simulink library "Lib_Piccolo"  (R2018b)
settings: Solver=VariableStepAuto  StartTime=0.0  StopTime=10.0  RelTol=1e-3
values from neighbouring files (symbols this model uses):
  AccelErrInt2Brakes = 0.15    [SimulationControlConfig16P.m]    (also in SimulationControlConfig16P_LEGACY.m; SimulationControlConfigTAILLESS.m = 0.2; SimulationControlConfigUTAIL.m = 0.2)
  AileronMax = 25    [SimulationControlConfig16P.m]    (also in SimulationControlConfig16P_LEGACY.m; SimulationControlConfigTAILLESS.m; SimulationControlConfigUTAIL.m)
  AileronPower = 0.00268    [SimulationControlConfig16P.m]    (also in SimulationControlConfig16P_LEGACY.m; SimulationControlConfigTAILLESS.m; SimulationControlConfigUTAIL.m)
  AileronSurfaceMax = 45    [SimulationControlConfig16P.m]    (also in SimulationControlConfig16P_LEGACY.m)
  AileronTrim = 0    [SimulationControlConfig16P.m]    (also in SimulationControlConfig16P_LEGACY.m; SimulationControlConfigTAILLESS.m; SimulationControlConfigUTAIL.m)
  Alt = 1000 + TerrainHeight    [SimulationStateConfig.m]
  AltCruise_m = testPlans(testIndx).terrainElevation * 0.3048 + 200    [SimulationControlConfig16P.m]    (also in SimulationControlConfigTAILLESS.m = 1083; SimulationControlConfigUTAIL.m = testPlans(testIndx).terrainElevation * 0.3048 + 152)
  AltitudeRate2PitchCmdIntegratorInit = 0.1    [SimulationControlPre.m]
  AltMax = 10000    [SimulationControlConfig16P.m]    (also in SimulationControlConfig16P_LEGACY.m; SimulationControlConfigTAILLESS.m; SimulationControlConfigUTAIL.m)
  AltMaxAccel = 1.25    [SimulationControlConfig16P.m]    (also in SimulationControlConfig16P_LEGACY.m = 0.9; SimulationControlConfigTAILLESS.m = 1.7; SimulationControlConfigUTAIL.m = 2)
  AltMin = 0    [SimulationControlConfig16P.m]    (also in SimulationControlConfig16P_LEGACY.m; SimulationControlConfigTAILLESS.m; SimulationControlConfigUTAIL.m)
  AltRateCmd2Pitch = 0.50    (= 0.5)    [SimulationControlConfig16P.m]    (also in SimulationControlConfig16P_LEGACY.m = 0.6; SimulationControlConfigTAILLESS.m = 0.2; SimulationControlConfigUTAIL.m = 0.3)
  AltRateError2Pitch = 0.40    (= 0.4)    [SimulationControlConfig16P.m]    (also in SimulationControlConfig16P_LEGACY.m; SimulationControlConfigTAILLESS.m = 0.55; SimulationControlConfigUTAIL.m = 0.55)
  AltRateErrorInt2Pitch = 0.50    (= 0.5)    [SimulationControlConfig16P.m]    (also in SimulationControlConfig16P_LEGACY.m = 0.45; SimulationControlConfigTAILLESS.m; SimulationControlConfigUTAIL.m = 0.75)
  AltRateLpfCutOff = 3    [SimulationControlConfig16P.m]    (also in SimulationControlConfig16P_LEGACY.m; SimulationControlConfigTAILLESS.m = 2; SimulationControlConfigUTAIL.m = 2)
  AutoNosegear2Rudder = 26    [SimulationControlConfig16P.m]    (also in SimulationControlConfig16P_LEGACY.m; SimulationControlConfigTAILLESS.m = 25.2; SimulationControlConfigUTAIL.m = 14)
  b = 5.54    [SimulationControlConfig16P.m]    (also in SimulationControlConfig16P_LEGACY.m; SimulationControlConfigTAILLESS.m = 2.37; SimulationControlConfigUTAIL.m = 2.37)
  Bank2AileronIntegratorInit = 0    [SimulationControlPre.m]
  BankMax_User = BankMax_User/180*pi    (= 0.523598775598)    [SimulationControlConfig16P.m]    (also in SimulationControlConfig16P_LEGACY.m; SimulationControlConfigTAILLESS.m = 0.610865238198; SimulationControlConfigUTAIL.m = 0.628318530718)
  baseLegFlaps = 20    [SimulationControlConfig16P.m]    (also in SimulationControlConfig16P_LEGACY.m = 0; SimulationControlConfigTAILLESS.m = 15; SimulationControlConfigUTAIL.m = 10)
  C = GeneticOpt.C    [SimulationCostFunction.m]
  c = Sw/b    (= 0.841696750903)    [SimulationControlConfig16P.m]    (also in SimulationControlConfig16P_LEGACY.m; SimulationControlConfigTAILLESS.m = 0.354008438819; SimulationControlConfigUTAIL.m = 0.354008438819)
  cell2WheelFactorMG = 5.98    [SimulationSensorConfig16P_LEGACY.m]
  cell2WheelFactorNG = 1    [SimulationSensorConfig16P_LEGACY.m]
  cellSatMaxMG = 15000    [SimulationSensorConfig16P.m]    (also in SimulationSensorConfig16P_LEGACY.m; SimulationSensorConfigTAILLESS7P.m; SimulationSensorConfigUTAIL7P.m)
  cellSatMaxNG = 1000    [SimulationSensorConfig16P.m]    (also in SimulationSensorConfig16P_LEGACY.m; SimulationSensorConfigTAILLESS7P.m; SimulationSensorConfigUTAIL7P.m)
  cellSatMinMG = -15000    [SimulationSensorConfig16P.m]    (also in SimulationSensorConfig16P_LEGACY.m; SimulationSensorConfigTAILLESS7P.m; SimulationSensorConfigUTAIL7P.m)
  cellSatMinNG = -1000    [SimulationSensorConfig16P.m]    (also in SimulationSensorConfig16P_LEGACY.m; SimulationSensorConfigTAILLESS7P.m; SimulationSensorConfigUTAIL7P.m)
  CL_Limit = CL_Max    (= 0.54)    [SimulationControlConfig16P.m]    (also in SimulationControlConfig16P_LEGACY.m; SimulationControlConfigTAILLESS.m; SimulationControlConfigUTAIL.m = 0.53)
  CL_Max = 0.54    [SimulationControlConfig16P.m]    (also in SimulationControlConfig16P_LEGACY.m; SimulationControlConfigTAILLESS.m; SimulationControlConfigUTAIL.m = 0.53)
  CL_Max_Nom = 0.465    [SimulationControlConfig16P.m]    (also in SimulationControlConfig16P_LEGACY.m; SimulationControlConfigTAILLESS.m = 0.39; SimulationControlConfigUTAIL.m)
  CL_Min = 0    [SimulationControlConfig16P.m]    (also in SimulationControlConfig16P_LEGACY.m; SimulationControlConfigTAILLESS.m; SimulationControlConfigUTAIL.m)
  ClimbMaxFraction = 0.35    [SimulationControlConfig16P.m]    (also in SimulationControlConfig16P_LEGACY.m = 0.24; SimulationControlConfigTAILLESS.m = 0.19; SimulationControlConfigUTAIL.m = 0.21)
  ClimboutMaxBank = 7.0    (= 7)    [SimulationControlConfig16P.m]    (also in SimulationControlConfig16P_LEGACY.m; SimulationControlConfigTAILLESS.m = 5; SimulationControlConfigUTAIL.m)
  ClimboutTimer = 7.0    (= 7)    [SimulationControlConfig16P.m]    (also in SimulationControlConfig16P_LEGACY.m; SimulationControlConfigTAILLESS.m; SimulationControlConfigUTAIL.m)
  dCl_per_dFlap = 0.005581818    [SimulationControlConfig16P.m]    (also in SimulationControlConfig16P_LEGACY.m = 0; SimulationControlConfigTAILLESS.m = 0; SimulationControlConfigUTAIL.m = 0)
  DecelerationCmd = 3.1    [SimulationControlConfig16P.m]    (also in SimulationControlConfig16P_LEGACY.m; SimulationControlConfigTAILLESS.m = 0.1; SimulationControlConfigUTAIL.m = 0.1)
  DeRotateLogicEndTimer = abs((NoseDownLimit_Deg-1)/DeRotateRamp_Dps)    [SimulationControlConfig16P.m]    (also in SimulationControlConfig16P_LEGACY.m; SimulationControlConfigTAILLESS.m; SimulationControlConfigUTAIL.m)
  DeRotateLogicHoldNoseUpTimer = 0.1    [SimulationControlConfig16P.m]    (also in SimulationControlConfig16P_LEGACY.m; SimulationControlConfigTAILLESS.m; SimulationControlConfigUTAIL.m)
  DeRotateLogicTimerTimeout = 2    [SimulationControlConfig16P.m]    (also in SimulationControlConfig16P_LEGACY.m; SimulationControlConfigTAILLESS.m; SimulationControlConfigUTAIL.m)
  DeRotateLowerCmdSaturation = 0    [SimulationControlConfig16P.m]    (also in SimulationControlConfig16P_LEGACY.m; SimulationControlConfigTAILLESS.m; SimulationControlConfigUTAIL.m)
  DeRotateRamp_Dps = 3    [SimulationControlConfig16P.m]    (also in SimulationControlConfig16P_LEGACY.m; SimulationControlConfigTAILLESS.m = 8; SimulationControlConfigUTAIL.m = 8)
  DeRotateUpperCmdSaturation = 7    [SimulationControlConfig16P.m]    (also in SimulationControlConfig16P_LEGACY.m; SimulationControlConfigTAILLESS.m; SimulationControlConfigUTAIL.m)
  DescentMaxFraction = 0.22    [SimulationControlConfig16P.m]    (also in SimulationControlConfig16P_LEGACY.m = 0.2; SimulationControlConfigTAILLESS.m = 0.17; SimulationControlConfigUTAIL.m = 0.17)
  DesktopSimTerrainOffset_m = 0.406    [SimulationAircraftConfig.m]
  downwindFlaps = 0    [SimulationControlConfig16P.m]    (also in SimulationControlConfig16P_LEGACY.m; SimulationControlConfigTAILLESS.m; SimulationControlConfigUTAIL.m)
  DP_init = 0.5*1.225*V_init^2    [SimulationControlConfig16P.m]    (also in SimulationControlConfig16P_LEGACY.m; SimulationControlConfigTAILLESS.m; SimulationControlConfigUTAIL.m)
  dscNoiseMG = 1    [SimulationSensorConfig16P_LEGACY.m]
  dscNoiseNG = 0.25    [SimulationSensorConfig16P_LEGACY.m]
  DSCnumBits = 24    [SimulationSensorConfig16P.m]    (also in SimulationSensorConfig16P_LEGACY.m; SimulationSensorConfigTAILLESS7P.m; SimulationSensorConfigUTAIL7P.m)
  DSCRangeMaxMG = 15000    [SimulationSensorConfig16P.m]    (also in SimulationSensorConfig16P_LEGACY.m; SimulationSensorConfigTAILLESS7P.m; SimulationSensorConfigUTAIL7P.m)
  DSCRangeMaxNG = 1000    [SimulationSensorConfig16P.m]    (also in SimulationSensorConfig16P_LEGACY.m; SimulationSensorConfigTAILLESS7P.m; SimulationSensorConfigUTAIL7P.m)
  DSCRangeMinMG = -15000    [SimulationSensorConfig16P.m]    (also in SimulationSensorConfig16P_LEGACY.m; SimulationSensorConfigTAILLESS7P.m; SimulationSensorConfigUTAIL7P.m)
  DSCRangeMinNG = -1000    [SimulationSensorConfig16P.m]    (also in SimulationSensorConfig16P_LEGACY.m; SimulationSensorConfigTAILLESS7P.m; SimulationSensorConfigUTAIL7P.m)
  dt = DLLSim.dt    [SimulationTimeStep.m]    (also in SimulationTrim.m = 0.02)
  EarlyTouchdownThreshold = 3.0    (= 3)    [SimulationControlConfig16P.m]    (also in SimulationControlConfig16P_LEGACY.m; SimulationControlConfigTAILLESS.m = 2.2; SimulationControlConfigUTAIL.m = 2.5)
  ElevatorDeflectionRate = 15    [SimulationControlConfig16P.m]    (also in SimulationControlConfig16P_LEGACY.m = 12; SimulationControlConfigTAILLESS.m = 10; SimulationControlConfigUTAIL.m = 12)
  ElevatorMax = 25    [SimulationControlConfig16P.m]    (also in SimulationControlConfig16P_LEGACY.m; SimulationControlConfigTAILLESS.m; SimulationControlConfigUTAIL.m)
  ElevatorPower = -0.002209    [SimulationControlConfig16P.m]    (also in SimulationControlConfig16P_LEGACY.m; SimulationControlConfigTAILLESS.m = -0.002956; SimulationControlConfigUTAIL.m = -0.00205983)
  ElevatorTrim = -3.5    [SimulationControlConfig16P.m]    (also in SimulationControlConfig16P_LEGACY.m; SimulationControlConfigTAILLESS.m = -6; SimulationControlConfigUTAIL.m = -8)
  elevonBias = 0    [SimulationControlConfig16P.m]    (also in SimulationControlConfig16P_LEGACY.m; SimulationControlConfigTAILLESS.m; SimulationControlConfigUTAIL.m)
  Enable_TAS_Protection = 0    [SimulationControlConfig16P.m]    (also in SimulationControlConfig16P_LEGACY.m; SimulationControlConfigTAILLESS.m; SimulationControlConfigUTAIL.m)
  EnableCrossTrackAbort = 1    [SimulationControlConfig16P.m]    (also in SimulationControlConfigTAILLESS.m; SimulationControlConfigUTAIL.m)
  EnergyBandwidth = 0.02    [SimulationControlConfig16P.m]    (also in SimulationControlConfig16P_LEGACY.m; SimulationControlConfigTAILLESS.m = 0.06; SimulationControlConfigUTAIL.m = 0.06)
  EngineLhFuelCut = 0    [SimulationAircraftConfig.m]
  EngineRhFuelCut = 0    [SimulationAircraftConfig.m]
  FastThrottleRate = 0.075    [SimulationControlConfig16P.m]    (also in SimulationControlConfig16P_LEGACY.m = 0.05; SimulationControlConfigTAILLESS.m = 0.1; SimulationControlConfigUTAIL.m = 0.1)
  FilterWarmUpTime = 2    [SimulationSensorConfig16P.m]    (also in SimulationSensorConfig16P_LEGACY.m; SimulationSensorConfigTAILLESS7P.m; SimulationSensorConfigUTAIL7P.m)
  finalApproachFlaps = 20    [SimulationControlConfig16P.m]    (also in SimulationControlConfig16P_LEGACY.m = 0; SimulationControlConfigTAILLESS.m = 22; SimulationControlConfigUTAIL.m = 10)
  FinalDescentSlope_Deg = testPlans(testIndx).descentSlope    [SimulationControlConfig16P.m]    (also in SimulationControlConfig16P_LEGACY.m; SimulationControlConfigTAILLESS.m; SimulationControlConfigUTAIL.m)
  flapMax = 0    [SimulationControlConfig16P.m]    (also in SimulationControlConfig16P_LEGACY.m; SimulationControlConfigTAILLESS.m; SimulationControlConfigUTAIL.m)
  flapRate = 7.5    [SimulationControlConfig16P.m]    (also in SimulationControlConfig16P_LEGACY.m; SimulationControlConfigTAILLESS.m = 6.6; SimulationControlConfigUTAIL.m)
  FlareHeight = 5    [SimulationControlConfig16P.m]    (also in SimulationControlConfig16P_LEGACY.m = 4.8; SimulationControlConfigTAILLESS.m = 2.5; SimulationControlConfigUTAIL.m = 2)
  FlareVerticalRate_mps = -0.4    [SimulationControlConfig16P.m]    (also in SimulationControlConfig16P_LEGACY.m = -0.5; SimulationControlConfigTAILLESS.m = -0.15; SimulationControlConfigUTAIL.m = -0.15)
  Fp_Aileron = 0.55*2*pi*RollRateLpfCutoff*dt    [SimulationControlConfig16P.m]    (also in SimulationControlConfig16P_LEGACY.m; SimulationControlConfigTAILLESS.m; SimulationControlConfigUTAIL.m)
  Fp_Alt = 0.55*AltBandwidth    (= 0.099)    [SimulationControlConfig16P.m]    (also in SimulationControlConfig16P_LEGACY.m; SimulationControlConfigTAILLESS.m = 0.587477826221; SimulationControlConfigUTAIL.m = 0.69115038379)
  Fp_AltRate = 0.55*2*pi*AltRateLpfCutOff*dt    [SimulationControlConfig16P.m]    (also in SimulationControlConfig16P_LEGACY.m; SimulationControlConfigTAILLESS.m; SimulationControlConfigUTAIL.m)
  Fp_Elevator = 0.55*2*pi*PitchRateLpfCutoff*dt    [SimulationControlConfig16P.m]    (also in SimulationControlConfig16P_LEGACY.m; SimulationControlConfigTAILLESS.m; SimulationControlConfigUTAIL.m)
  Fp_Energy = 0.55*2*pi*EnergyBandwidth    (= 0.069115038379)    [SimulationControlConfig16P.m]    (also in SimulationControlConfig16P_LEGACY.m; SimulationControlConfigTAILLESS.m = 0.207345115137; SimulationControlConfigUTAIL.m = 0.207345115137)
  Fp_Energy2 = 0.55*2*pi*EnergyBandwidth*dt    [SimulationControlConfig16P.m]    (also in SimulationControlConfig16P_LEGACY.m; SimulationControlConfigTAILLESS.m; SimulationControlConfigUTAIL.m)
  Fp_Pitch = 0.55*2*pi*PitchBandwidth    (= 2.76460153516)    [SimulationControlConfig16P.m]    (also in SimulationControlConfig16P_LEGACY.m = 3.11017672705; SimulationControlConfigTAILLESS.m = 3.80132711084; SimulationControlConfigUTAIL.m = 2.41902634326)
  Fp_Pitch_2 = 0.55*2*pi*PitchBandwidth*dt    [SimulationControlConfig16P.m]    (also in SimulationControlConfig16P_LEGACY.m; SimulationControlConfigTAILLESS.m; SimulationControlConfigUTAIL.m)
  Fp_Roll = RollBandwidth^2    (= 1)    [SimulationControlConfig16P.m]    (also in SimulationControlConfig16P_LEGACY.m = 1.44; SimulationControlConfigTAILLESS.m; SimulationControlConfigUTAIL.m)
  Fp_Rudder = 0.55*2*pi*YawRateLpfCutoff*dt    [SimulationControlConfig16P.m]    (also in SimulationControlConfig16P_LEGACY.m; SimulationControlConfigTAILLESS.m; SimulationControlConfigUTAIL.m)
  Fp_TAS = 0.55*2*pi*TASBandwidth    (= 0.103672557568)    [SimulationControlConfig16P.m]    (also in SimulationControlConfig16P_LEGACY.m; SimulationControlConfigTAILLESS.m = 0.172787595947; SimulationControlConfigUTAIL.m = 0.172787595947)
  Fp_TAS_Filter = 2*pi*TasLpfCutoff*dt    [SimulationControlConfig16P.m]    (also in SimulationControlConfig16P_LEGACY.m; SimulationControlConfigTAILLESS.m; SimulationControlConfigUTAIL.m)
  Fp_Turn = 0.55*2*pi*TurnErrLPFcutoff    (= 0.0345575191895)    [SimulationControlConfig16P.m]    (also in SimulationControlConfig16P_LEGACY.m; SimulationControlConfigTAILLESS.m = 0.172787595947; SimulationControlConfigUTAIL.m = 0.172787595947)
  Fp_TurnDerr = 0.55*2*pi*TurnDerivativeLPFcutoff    (= 0.0345575191895)    [SimulationControlConfig16P.m]    (also in SimulationControlConfig16P_LEGACY.m; SimulationControlConfigTAILLESS.m = 0.172787595947; SimulationControlConfigUTAIL.m = 0.172787595947)
  FTV = 3    [SimulationAircraftConfig.m]
  ftvStaticPositionError = 1/1.18    (= 0.847457627119)    [SimulationSensorConfig16P.m]    (also in SimulationSensorConfig16P_LEGACY.m; SimulationSensorConfigTAILLESS7P.m = 1; SimulationSensorConfigUTAIL7P.m = 1)
  g = 9.81    [SimulationStateConfig.m]
  GustSpd_Kts = testPlans(testIndx).gustSpd    [SimulationStateConfig.m]
  GustTriggerVal = testPlans(testIndx).gustTriggerVal    [SimulationStateConfig.m]
  HeadingErr2TurnRate = 0.5    [SimulationControlConfig16P.m]    (also in SimulationControlConfig16P_LEGACY.m; SimulationControlConfigTAILLESS.m; SimulationControlConfigUTAIL.m)
  HeadingErrDer2TurnRate = 0.3    [SimulationControlConfig16P.m]    (also in SimulationControlConfig16P_LEGACY.m; SimulationControlConfigTAILLESS.m; SimulationControlConfigUTAIL.m)
  IASbounce = IASstall*0.8    [SimulationControlPre.m]
  IAScruiseCMD = sqrt(2*m*9.81/(1.225*Sw*CL_cruise))    [SimulationControlConfig16P.m]    (also in SimulationControlConfig16P_LEGACY.m; SimulationControlConfigTAILLESS.m; SimulationControlConfigUTAIL.m)
  IASfinalCMD = 1.12 * IASmin    [SimulationControlConfig16P.m]    (also in SimulationControlConfig16P_LEGACY.m = 1.10 * IASmin; SimulationControlConfigTAILLESS.m = 1.10 * IASmin; SimulationControlConfigUTAIL.m = 1.15 * IASmin)
  IASflareCMD = IASstall    [SimulationControlConfig16P.m]    (also in SimulationControlConfig16P_LEGACY.m; SimulationControlConfigTAILLESS.m; SimulationControlConfigUTAIL.m)
  IASmax = 64    [SimulationControlConfig16P.m]    (also in SimulationControlConfig16P_LEGACY.m = 46; SimulationControlConfigTAILLESS.m = 38.58; SimulationControlConfigUTAIL.m = 35)
  IASmin = sqrt(2*m*9.81/(1.225*Sw*0.9*CL_Max_Nom))    [SimulationControlConfig16P.m]    (also in SimulationControlConfig16P_LEGACY.m; SimulationControlConfigTAILLESS.m; SimulationControlConfigUTAIL.m)
  IASshortCMD = IASstall    [SimulationControlConfig16P.m]    (also in SimulationControlConfig16P_LEGACY.m; SimulationControlConfigTAILLESS.m; SimulationControlConfigUTAIL.m)
  IASstall = sqrt(2*m*9.81/(1.225*Sw*CL_Max))    [SimulationControlConfig16P.m]    (also in SimulationControlConfig16P_LEGACY.m; SimulationControlConfigTAILLESS.m; SimulationControlConfigUTAIL.m)
  inFlight = 1    [SimulationControlConfig16P.m]    (also in SimulationControlConfigTAILLESS.m; SimulationControlConfigUTAIL.m)
  JetCatOffset = 5    [SimulationControlConfig16P.m]    (also in SimulationControlConfig16P_LEGACY.m)
  LaunchRollingElevator = -1.5    [SimulationControlConfig16P.m]    (also in SimulationControlConfig16P_LEGACY.m; SimulationControlConfigTAILLESS.m = 1; SimulationControlConfigUTAIL.m = 1)
  ldg_NosegearMax = 10    [SimulationControlConfig16P.m]    (also in SimulationControlConfig16P_LEGACY.m; SimulationControlConfigTAILLESS.m; SimulationControlConfigUTAIL.m)
  ldg_TrackVyErrInt2Nosegear = 0.1250    (= 0.125)    [SimulationControlConfig16P.m]    (also in SimulationControlConfig16P_LEGACY.m; SimulationControlConfigTAILLESS.m = 0.00714285714286; SimulationControlConfigUTAIL.m = 0.00714285714286)
  ldg_TrackVyErrPro2Nosegear = 0.35    [SimulationControlConfig16P.m]    (also in SimulationControlConfig16P_LEGACY.m; SimulationControlConfigTAILLESS.m = 0.0546666666667; SimulationControlConfigUTAIL.m = 0.0546666666667)
  ldg_TrackY2Vy = 0.07    [SimulationControlConfig16P.m]    (also in SimulationControlConfig16P_LEGACY.m; SimulationControlConfigTAILLESS.m = 0.17; SimulationControlConfigUTAIL.m = 0.17)
  ldg_Vy2NosegearScalingPower = 1.075    [SimulationControlConfig16P.m]    (also in SimulationControlConfig16P_LEGACY.m; SimulationControlConfigTAILLESS.m = 0.6; SimulationControlConfigUTAIL.m = 0.5)
  ldg_Y2VyScalingPower = 0.175    [SimulationControlConfig16P.m]    (also in SimulationControlConfig16P_LEGACY.m; SimulationControlConfigTAILLESS.m = 0; SimulationControlConfigUTAIL.m = 0)
  ldg_YawRate2Nosegear = 0.175    [SimulationControlConfig16P.m]    (also in SimulationControlConfig16P_LEGACY.m; SimulationControlConfigTAILLESS.m = 0.065; SimulationControlConfigUTAIL.m = 0.065)
  LiftSlope = 0.064285    [SimulationControlConfig16P.m]    (also in SimulationControlConfig16P_LEGACY.m; SimulationControlConfigTAILLESS.m = 0.058631; SimulationControlConfigUTAIL.m)
  LPFaileronInit = 0    [SimulationControlPre.m]
  LPFclestInit = 0    [SimulationControlPre.m]
  LPFenergyFFInit = 0    [SimulationControlPre.m]
  LPFtasInit = V_init + 2    [SimulationControlPre.m]
  LPFthrottleInit = ThrottleTrim    [SimulationControlPre.m]
  LPFturnErrInit = 0    [SimulationControlPre.m]
  ... (+115 more)
undefined symbols (not defined in the file or in its folder): abortFlag, alphaHPF, apmDelay, BRWNOUT, CRAWOR, CRAWUR, DiscIntNeverNeededParam, DLLSim, DLLSimStep, ECOMOR, ECOMUR, Fp_Tas, GustTrigger_HeightAgl_m, IPSTAT, LCINTEG, Ldg_Persist_Time, LOWER_FLAGS, MSG_ENABLE, NoiseStd, OLDVAL, OVERRIDE_ENABLE, OVERRIDE_VALUE, REBOOT, reversionEnable, revIASMax, revIASMin, revPitchMax, revPitchMin, revPitchRateMax, revRollMax, revRollRateMax, SAMPLE, SCALON, SensorModel, sigbuilder_block, Sim_Vx, Sim_Vy, Sim_Vz, Sim_Xpos, Sim_Ypos, Sim_Zpos, SYSOR, SYSUR, TARE, TEMPOR, TEMPUR, testIndx, testPlan, testPlans, Trim_piccoloInCmd, Trim_REFSI_FD_IN_nmodeCgShifterCmd_Ft, Trim_REFSI_FD_IN_nmodeFlapLhIBCmd_Deg, Trim_REFSI_FD_IN_nmodeFlapLhOBCmd_Deg, Trim_REFSI_FD_IN_nmodeFlapRhIBCmd_Deg, Trim_REFSI_FD_IN_nmodeFlapRhOBCmd_Deg, Trim_REFSI_FD_IN_nmodeSlatLhCmd_Deg, Trim_REFSI_FD_IN_nmodeSlatRhCmd_Deg, Trim_REFSI_FD_IN_nmodeSplrLhInbdCmd_Deg, Trim_REFSI_FD_IN_nmodeSplrLhOutbdCmd_Deg ... (+5)
libraries: simulink x866, aerolibconvert2 x60, $bdroot x52, aerolibatmos2 x5, dspswit3 x5, simulink_extras x4, dsparch4 x2, Lib_Piccolo_Alt x2, eeGeneralControl x1, dspindex x1
(part 24 of 44)

== system Lib_Piccolo/WOW Archive Container/Load Cell WoW Model 4 - LiftOff Delay variation 2/T//O Configuration ==
  note: Unlike when landing our persistance and latching is inverted relative to Weight Off both gears.
      |
      | Protection against WOW Failure. In the Event of a Sensor Failure and AC lift's off, NZ threshold overides WOW signal.
  Sim.WOW_Filt : Inport
  AND : Logic  IconShape=distinctive  AllPortsSameDT=off  OutDataTypeStr=boolean
  Bus Selector : BusSelector  OutputSignals=Sim:WOW_Filt_NG,Sim:WOW_Filt_L,Sim:WOW_Filt_R
  Compare To Constant1 : simulink/Logic and Bit Operations/Compare To Constant  relop=<  const=TO_Load_Thresh  OutDataTypeStr=uint8
  Compare To Constant2 : simulink/Logic and Bit Operations/Compare To Constant  relop=<  const=TO_Load_Thresh  OutDataTypeStr=uint8
  Latch : Subsystem
  Latch Timer : Subsystem  mask{period=TO_Latch_Time}
      mask prompts: period "Period [s]"
  NOT : Logic  Operator=NOT  IconShape=distinctive  AllPortsSameDT=off  OutDataTypeStr=boolean
  NOT2 : Logic  Operator=NOT  IconShape=distinctive  AllPortsSameDT=off  OutDataTypeStr=boolean
  Persistance Timer : Subsystem  mask{period=TO_Persist_Time}
      mask prompts: period "Period [s]"
  Terminator : Terminator
  Unit Delay : UnitDelay  SampleTime=-1
  ContactBool : Outport
  wires:
  NOT2/1 -> ContactBool/1
  Persistance Timer/1(Expired) -> Latch/1(D)
  Compare To Constant2/1 -> AND/1
  Latch Timer/1(Expired) -> NOT/1
  Unit Delay/1 -> Latch Timer/1(Enable/!Rst)
  Compare To Constant1/1 -> AND/2
  AND/1 -> Persistance Timer/1(Enable/!Rst)
  Latch/1(Q_Latched) -> Unit Delay/1, NOT2/1  "ContactBool"
  NOT/1 -> Latch/2(Enable/!Rst)
  Sim.WOW_Filt/1 -> Bus Selector/1
  Bus Selector/1 -> Terminator/1  "<Sim:WOW_Filt_NG>"
  Bus Selector/2 -> Compare To Constant2/1  "<Sim:WOW_Filt_L>"
  Bus Selector/3 -> Compare To Constant1/1  "<Sim:WOW_Filt_R>"

== system Lib_Piccolo/WOW Archive Container/Load Cell WoW Model 5 - Dynamic Timing/LPF L ==
  Input : Inport
  Reset : Inport  Port=2
  Add1 : Sum  Inputs=++|
  Compare To Constant2 : simulink/Logic and Bit Operations/Compare To Constant  relop=>  const=0  OutDataTypeStr=uint8
  Constant11 : Constant  Value=Cutoff
  Switch1 : Switch  Criteria=u2 > Threshold
  Unit Delay1 : UnitDelay  InitialCondition=Init  SampleTime=-1
  a1 : Gain  Gain=SensorModel.WOW.Cell.a1
  b0 : Gain  Gain=SensorModel.WOW.Cell.b0
  Output : Outport
  wires:
  Constant11/1 -> Compare To Constant2/1
  Compare To Constant2/1 -> Switch1/2
  Switch1/1 -> Output/1
  Input/1 -> b0/1, Switch1/3
  a1/1 -> Add1/1
  Add1/1 -> Switch1/1, Unit Delay1/1
  b0/1 -> Add1/2
  Unit Delay1/1 -> a1/1

== system Lib_Piccolo/WOW Archive Container/Load Cell WoW Model 5 - Dynamic Timing/LPF N ==
  Input : Inport
  Reset : Inport  Port=2
  Add1 : Sum  Inputs=++|
  Compare To Constant2 : simulink/Logic and Bit Operations/Compare To Constant  relop=>  const=0  OutDataTypeStr=uint8
  Constant11 : Constant  Value=Cutoff
  Switch1 : Switch  Criteria=u2 > Threshold
  Unit Delay1 : UnitDelay  InitialCondition=Init  SampleTime=-1
  a1 : Gain  Gain=SensorModel.WOW.Cell.a1
  b0 : Gain  Gain=SensorModel.WOW.Cell.b0
  Output : Outport
  wires:
  Constant11/1 -> Compare To Constant2/1
  Compare To Constant2/1 -> Switch1/2
  Switch1/1 -> Output/1
  Input/1 -> b0/1, Switch1/3
  a1/1 -> Add1/1
  Add1/1 -> Switch1/1, Unit Delay1/1
  b0/1 -> Add1/2
  Unit Delay1/1 -> a1/1

== system Lib_Piccolo/WOW Archive Container/Load Cell WoW Model 5 - Dynamic Timing/LPF R ==
  Input : Inport
  Reset : Inport  Port=2
  Add1 : Sum  Inputs=++|
  Compare To Constant2 : simulink/Logic and Bit Operations/Compare To Constant  relop=>  const=0  OutDataTypeStr=uint8
  Constant11 : Constant  Value=Cutoff
  Switch1 : Switch  Criteria=u2 > Threshold
  Unit Delay1 : UnitDelay  InitialCondition=Init  SampleTime=-1
  a1 : Gain  Gain=SensorModel.WOW.Cell.a1
  b0 : Gain  Gain=SensorModel.WOW.Cell.b0
  Output : Outport
  wires:
  Constant11/1 -> Compare To Constant2/1
  Compare To Constant2/1 -> Switch1/2
  Switch1/1 -> Output/1
  Input/1 -> b0/1, Switch1/3
  a1/1 -> Add1/1
  Add1/1 -> Switch1/1, Unit Delay1/1
  b0/1 -> Add1/2
  Unit Delay1/1 -> a1/1

== system Lib_Piccolo/WOW Archive Container/Load Cell WoW Model 5 - Dynamic Timing/Landing Configuration ==
  Sim.WOW_Filt : Inport
  Piccolo AP Mode : Inport  Port=2
  " Dynamic Timer" : $bdroot/ Dynamic Timer
  AND : Logic  IconShape=distinctive  AllPortsSameDT=off  OutDataTypeStr=boolean
  AND1 : Logic  IconShape=distinctive  AllPortsSameDT=off  OutDataTypeStr=boolean
  AND4 : Logic  IconShape=distinctive  AllPortsSameDT=off  OutDataTypeStr=boolean
  Bus Selector : BusSelector  OutputSignals=Sim:WOW_Filt_NG,Sim:WOW_Filt_L,Sim:WOW_Filt_R
  Compare To Constant : simulink/Logic and Bit Operations/Compare To Constant  relop=>  const=9  OutDataTypeStr=boolean
  Gain1 : Gain
  Gain2 : Gain
  Hysteresis L : Relay  OnSwitchValue=Ldg_Load_Thresh_Upper  OffSwitchValue=Ldg_Load_Thresh_Lower
  Hysteresis R : Relay  OnSwitchValue=Ldg_Load_Thresh_Upper  OffSwitchValue=Ldg_Load_Thresh_Lower
  Latch : Subsystem
  Latch Timer Selection : Subsystem
  NOT : Logic  Operator=NOT  IconShape=distinctive  AllPortsSameDT=off  OutDataTypeStr=boolean
  NOT2 : Logic  Operator=NOT  IconShape=distinctive  AllPortsSameDT=off  OutDataTypeStr=boolean
  OR1 : Logic  Operator=OR  IconShape=distinctive  AllPortsSameDT=off  OutDataTypeStr=boolean
  Persistance Timer Initial Touchdown : Subsystem  mask{period=Ldg_Persist_Time}
      mask prompts: period "Period [s]"
  TImer Period Selection : Subsystem
  Terminator : Terminator
  Terminator1 : Terminator
  Terminator2 : Terminator
  detectionLatch : Subsystem
  ContactBool : Outport
  tag scope: apModeEnable=global, hasDetected=global
  wires:
  Compare To Constant/1 -> [apModeEnable]
  Piccolo AP Mode/1 -> Compare To Constant/1
  detectionLatch/1(Q_Latched) -> [hasDetected]  "hasDetected"
  [apModeEnable] -> detectionLatch/2(Enable/!Rst)
  Bus Selector/3 -> Hysteresis R/1, TImer Period Selection/2(WOW_RMG)  "<Sim:WOW_Filt_R>"
  Bus Selector/2 -> TImer Period Selection/1(WOW_LMG), Hysteresis L/1  "<Sim:WOW_Filt_L>"
  Bus Selector/1 -> Terminator/1  "<Sim:WOW_Filt_NG>"
  Sim.WOW_Filt/1 -> Bus Selector/1
  Latch/1(Q_Latched) -> detectionLatch/1(D), OR1/1, Latch Timer Selection/1(ContactBool)  "ContactBool"
  Gain2/1 -> Terminator2/1  "ContactR"
  Gain1/1 -> Terminator1/1  "ContactL"
  Hysteresis R/1 -> Gain2/1, AND/2
  Hysteresis L/1 -> Gain1/1, AND/1
  Latch Timer Selection/1(switchedTimer) -> Latch/2(Enable/!Rst)  "Touchdown_Latch_Reset"
  Persistance Timer Initial Touchdown/1(Expired) -> Latch/1(D)
  " Dynamic Timer"/1 -> NOT2/1  "PersistanceLiftOff"
  OR1/1 -> ContactBool/1
  NOT/1 -> AND4/1
  AND4/1 -> " Dynamic Timer"/1
  [hasDetected] -> AND4/2, AND1/2
  NOT2/1 -> AND1/1
  AND/1 -> NOT/1, Persistance Timer Initial Touchdown/1(Enable/!Rst)
  TImer Period Selection/1(Dynamic Timer Period) -> " Dynamic Timer"/2
  AND1/1 -> OR1/2

== system Lib_Piccolo/WOW Archive Container/Load Cell WoW Model 5 - Dynamic Timing/T//O Configuration ==
  note: Unlike when landing our persistance and latching is inverted relative to Weight Off both gears.
      |
      | Protection against WOW Failure. In the Event of a Sensor Failure and AC lift's off, NZ threshold overides WOW signal.
  Sim.WOW_Filt : Inport
  AND : Logic  IconShape=distinctive  AllPortsSameDT=off  OutDataTypeStr=boolean
  Bus Selector : BusSelector  OutputSignals=Sim:WOW_Filt_NG,Sim:WOW_Filt_L,Sim:WOW_Filt_R
  Compare To Constant1 : simulink/Logic and Bit Operations/Compare To Constant  relop=<  const=TO_Load_Thresh  OutDataTypeStr=uint8
  Compare To Constant2 : simulink/Logic and Bit Operations/Compare To Constant  relop=<  const=TO_Load_Thresh  OutDataTypeStr=uint8
  Latch : Subsystem
  Latch Timer : Subsystem  mask{period=TO_Latch_Time}
      mask prompts: period "Period [s]"
  NOT : Logic  Operator=NOT  IconShape=distinctive  AllPortsSameDT=off  OutDataTypeStr=boolean
  NOT2 : Logic  Operator=NOT  IconShape=distinctive  AllPortsSameDT=off  OutDataTypeStr=boolean
  Persistance Timer : Subsystem  mask{period=TO_Persist_Time}
      mask prompts: period "Period [s]"
  Terminator : Terminator
  Unit Delay : UnitDelay  SampleTime=-1
  ContactBool : Outport
  wires:
  Bus Selector/3 -> Compare To Constant1/1  "<Sim:WOW_Filt_R>"
  Bus Selector/2 -> Compare To Constant2/1  "<Sim:WOW_Filt_L>"
  Bus Selector/1 -> Terminator/1  "<Sim:WOW_Filt_NG>"
  Sim.WOW_Filt/1 -> Bus Selector/1
  NOT/1 -> Latch/2(Enable/!Rst)
  Latch/1(Q_Latched) -> NOT2/1, Unit Delay/1  "ContactBool"
  AND/1 -> Persistance Timer/1(Enable/!Rst)
  Compare To Constant1/1 -> AND/2
  Unit Delay/1 -> Latch Timer/1(Enable/!Rst)
  Latch Timer/1(Expired) -> NOT/1
  Compare To Constant2/1 -> AND/1
  Persistance Timer/1(Expired) -> Latch/1(D)
  NOT2/1 -> ContactBool/1

== system Lib_Piccolo/WOW Archive Container/Load Cell WoW Model 6 - LiftOff Delay variation 3/LPF L ==
  Input : Inport
  Reset : Inport  Port=2
  Add1 : Sum  Inputs=++|
  Compare To Constant2 : simulink/Logic and Bit Operations/Compare To Constant  relop=>  const=0  OutDataTypeStr=uint8
  Constant11 : Constant  Value=Cutoff
  Switch1 : Switch  Criteria=u2 > Threshold
  Unit Delay1 : UnitDelay  InitialCondition=Init  SampleTime=-1
  a1 : Gain  Gain=SensorModel.WOW.Cell.a1
  b0 : Gain  Gain=SensorModel.WOW.Cell.b0
  Output : Outport
  wires:
  Constant11/1 -> Compare To Constant2/1
  Compare To Constant2/1 -> Switch1/2
  Switch1/1 -> Output/1
  Input/1 -> b0/1, Switch1/3
  a1/1 -> Add1/1
  Add1/1 -> Switch1/1, Unit Delay1/1
  b0/1 -> Add1/2
  Unit Delay1/1 -> a1/1

== system Lib_Piccolo/WOW Archive Container/Load Cell WoW Model 6 - LiftOff Delay variation 3/LPF N ==
  Input : Inport
  Reset : Inport  Port=2
  Add1 : Sum  Inputs=++|
  Compare To Constant2 : simulink/Logic and Bit Operations/Compare To Constant  relop=>  const=0  OutDataTypeStr=uint8
  Constant11 : Constant  Value=Cutoff
  Switch1 : Switch  Criteria=u2 > Threshold
  Unit Delay1 : UnitDelay  InitialCondition=Init  SampleTime=-1
  a1 : Gain  Gain=SensorModel.WOW.Cell.a1
  b0 : Gain  Gain=SensorModel.WOW.Cell.b0
  Output : Outport
  wires:
  Constant11/1 -> Compare To Constant2/1
  Compare To Constant2/1 -> Switch1/2
  Switch1/1 -> Output/1
  Input/1 -> b0/1, Switch1/3
  a1/1 -> Add1/1
  Add1/1 -> Switch1/1, Unit Delay1/1
  b0/1 -> Add1/2
  Unit Delay1/1 -> a1/1

== system Lib_Piccolo/WOW Archive Container/Load Cell WoW Model 6 - LiftOff Delay variation 3/LPF R ==
  Input : Inport
  Reset : Inport  Port=2
  Add1 : Sum  Inputs=++|
  Compare To Constant2 : simulink/Logic and Bit Operations/Compare To Constant  relop=>  const=0  OutDataTypeStr=uint8
  Constant11 : Constant  Value=Cutoff
  Switch1 : Switch  Criteria=u2 > Threshold
  Unit Delay1 : UnitDelay  InitialCondition=Init  SampleTime=-1
  a1 : Gain  Gain=SensorModel.WOW.Cell.a1
  b0 : Gain  Gain=SensorModel.WOW.Cell.b0
  Output : Outport
  wires:
  Constant11/1 -> Compare To Constant2/1
  Compare To Constant2/1 -> Switch1/2
  Switch1/1 -> Output/1
  Input/1 -> b0/1, Switch1/3
  a1/1 -> Add1/1
  Add1/1 -> Switch1/1, Unit Delay1/1
  b0/1 -> Add1/2
  Unit Delay1/1 -> a1/1

== system Lib_Piccolo/WOW Archive Container/Load Cell WoW Model 6 - LiftOff Delay variation 3/Landing Configuration ==
  Sim.WOW_Filt : Inport
  Piccolo AP Mode : Inport  Port=2
  AND{,1..2,4} (4 alike) : Logic  IconShape=distinctive  AllPortsSameDT=off  OutDataTypeStr=boolean
  AND3 : Logic  Inputs=3  IconShape=distinctive  AllPortsSameDT=off  OutDataTypeStr=boolean
  Bus Selector : BusSelector  OutputSignals=Sim:WOW_Filt_NG,Sim:WOW_Filt_L,Sim:WOW_Filt_R
  Compare To Constant : simulink/Logic and Bit Operations/Compare To Constant  relop=>  const=9  OutDataTypeStr=boolean
  Gain : Gain
  Gain1 : Gain
  Gain2 : Gain
  Hysteresis L : Relay  OnSwitchValue=Ldg_Load_Thresh_Upper  OffSwitchValue=Ldg_Load_Thresh_Lower
  Hysteresis R : Relay  OnSwitchValue=Ldg_Load_Thresh_Upper  OffSwitchValue=Ldg_Load_Thresh_Lower
  LiftOff Double Wheel : Subsystem  mask{period=SensorModel.WOW.Cell.LiftOffLatchTimeDoubleWheel}
      mask prompts: period "Period [s]"
  LiftOff Single Wheel : Subsystem  mask{period=SensorModel.WOW.Cell.LiftOffLatchTimeSingleWheel}
      mask prompts: period "Period [s]"
  NOT{,1..3} (4 alike) : Logic  Operator=NOT  IconShape=distinctive  AllPortsSameDT=off  OutDataTypeStr=boolean
  OR : Logic  Operator=OR  IconShape=distinctive  AllPortsSameDT=off  OutDataTypeStr=boolean
  OR1 : Logic  Operator=OR  IconShape=distinctive  AllPortsSameDT=off  OutDataTypeStr=boolean
  OR2 : Logic  Operator=OR  IconShape=distinctive  AllPortsSameDT=off  OutDataTypeStr=boolean
  Persistance Timer Initial Touchdown : Subsystem  mask{period=Ldg_Persist_Time}
      mask prompts: period "Period [s]"
  Terminator : Terminator
  Terminator1 : Terminator
  Terminator2 : Terminator
  detectionLatch : Subsystem
  ContactBool : Outport
  tag scope: apModeEnable=global, hasDetected=global
  wires:
  AND3/1 -> OR2/1  "ContactBool-LiftOffPersistanceSingleWheelOff"
  [hasDetected] -> AND4/2, AND3/2
  NOT2/1 -> AND3/1
  AND4/1 -> LiftOff Single Wheel/1(Enable/!Rst)
  NOT/1 -> AND4/1
  OR1/1 -> ContactBool/1  "ContactBool"
  LiftOff Single Wheel/1(Expired) -> NOT2/1  "PersistanceLiftOff"
  Persistance Timer Initial Touchdown/1(Expired) -> detectionLatch/1(D), Gain/1
  Hysteresis L/1 -> OR/1, AND/1, Gain1/1
  Hysteresis R/1 -> OR/2, AND/2, Gain2/1
  Gain1/1 -> Terminator1/1  "ContactL"
  Gain2/1 -> Terminator2/1  "ContactR"
  Gain/1 -> OR1/1  "ContactBool-ActiveContact"
  Sim.WOW_Filt/1 -> Bus Selector/1
  Bus Selector/1 -> Terminator/1  "<Sim:WOW_Filt_NG>"
  Bus Selector/2 -> Hysteresis L/1  "<Sim:WOW_Filt_L>"
  Bus Selector/3 -> Hysteresis R/1  "<Sim:WOW_Filt_R>"
  [apModeEnable] -> detectionLatch/2(Enable/!Rst)
  detectionLatch/1(Q_Latched) -> [hasDetected]  "hasDetected"
  Piccolo AP Mode/1 -> Compare To Constant/1
  Compare To Constant/1 -> [apModeEnable]
  LiftOff Double Wheel/1(Expired) -> NOT3/1  "PersistanceLiftOff"
  NOT1/1 -> AND2/1
  [hasDetected] -> AND2/2, AND1/2
  AND1/1 -> OR2/2  "ContactBool-LiftOffPersistanceDoubleWheel"
  NOT3/1 -> AND1/1
  AND2/1 -> LiftOff Double Wheel/1(Enable/!Rst)
  AND/1 -> NOT/1, NOT1/1, Persistance Timer Initial Touchdown/1(Enable/!Rst)
  OR2/1 -> OR1/2  "ContactBool-LiftOffPersistance"
  OR/1 -> AND3/3

== system Lib_Piccolo/WOW Archive Container/Load Cell WoW Model 6 - LiftOff Delay variation 3/T//O Configuration ==
  note: Unlike when landing our persistance and latching is inverted relative to Weight Off both gears.
      |
      | Protection against WOW Failure. In the Event of a Sensor Failure and AC lift's off, NZ threshold overides WOW signal.
  Sim.WOW_Filt : Inport
  AND : Logic  IconShape=distinctive  AllPortsSameDT=off  OutDataTypeStr=boolean
  Bus Selector : BusSelector  OutputSignals=Sim:WOW_Filt_NG,Sim:WOW_Filt_L,Sim:WOW_Filt_R
  Compare To Constant1 : simulink/Logic and Bit Operations/Compare To Constant  relop=<  const=TO_Load_Thresh  OutDataTypeStr=uint8
  Compare To Constant2 : simulink/Logic and Bit Operations/Compare To Constant  relop=<  const=TO_Load_Thresh  OutDataTypeStr=uint8
  Latch : Subsystem
  Latch Timer : Subsystem  mask{period=TO_Latch_Time}
      mask prompts: period "Period [s]"
  NOT : Logic  Operator=NOT  IconShape=distinctive  AllPortsSameDT=off  OutDataTypeStr=boolean
  NOT2 : Logic  Operator=NOT  IconShape=distinctive  AllPortsSameDT=off  OutDataTypeStr=boolean
  Persistance Timer : Subsystem  mask{period=TO_Persist_Time}
      mask prompts: period "Period [s]"
  Terminator : Terminator
  Unit Delay : UnitDelay  SampleTime=-1
  ContactBool : Outport
  wires:
  Bus Selector/3 -> Compare To Constant1/1  "<Sim:WOW_Filt_R>"
  Bus Selector/2 -> Compare To Constant2/1  "<Sim:WOW_Filt_L>"
  Bus Selector/1 -> Terminator/1  "<Sim:WOW_Filt_NG>"
  Sim.WOW_Filt/1 -> Bus Selector/1
  NOT/1 -> Latch/2(Enable/!Rst)
  Latch/1(Q_Latched) -> NOT2/1, Unit Delay/1  "ContactBool"
  AND/1 -> Persistance Timer/1(Enable/!Rst)
  Compare To Constant1/1 -> AND/2
  Unit Delay/1 -> Latch Timer/1(Enable/!Rst)
  Latch Timer/1(Expired) -> NOT/1
  Compare To Constant2/1 -> AND/1
  Persistance Timer/1(Expired) -> Latch/1(D)
  NOT2/1 -> ContactBool/1

== system Lib_Piccolo/WOW Archive Container/Load Cell WoW Model 7 - LiftOff Delay variation 4/LPF L ==
  Input : Inport
  Reset : Inport  Port=2
  Add1 : Sum  Inputs=++|
  Compare To Constant2 : simulink/Logic and Bit Operations/Compare To Constant  relop=>  const=0  OutDataTypeStr=uint8
  Constant11 : Constant  Value=Cutoff
  Switch1 : Switch  Criteria=u2 > Threshold
  Unit Delay1 : UnitDelay  InitialCondition=Init  SampleTime=-1
  a1 : Gain  Gain=SensorModel.WOW.Cell.a1
  b0 : Gain  Gain=SensorModel.WOW.Cell.b0
  Output : Outport
  wires:
  Constant11/1 -> Compare To Constant2/1
  Compare To Constant2/1 -> Switch1/2
  Switch1/1 -> Output/1
  Input/1 -> b0/1, Switch1/3
  a1/1 -> Add1/1
  Add1/1 -> Switch1/1, Unit Delay1/1
  b0/1 -> Add1/2
  Unit Delay1/1 -> a1/1

== system Lib_Piccolo/WOW Archive Container/Load Cell WoW Model 7 - LiftOff Delay variation 4/LPF N ==
  Input : Inport
  Reset : Inport  Port=2
  Add1 : Sum  Inputs=++|
  Compare To Constant2 : simulink/Logic and Bit Operations/Compare To Constant  relop=>  const=0  OutDataTypeStr=uint8
  Constant11 : Constant  Value=Cutoff
  Switch1 : Switch  Criteria=u2 > Threshold
  Unit Delay1 : UnitDelay  InitialCondition=Init  SampleTime=-1
  a1 : Gain  Gain=SensorModel.WOW.Cell.a1
  b0 : Gain  Gain=SensorModel.WOW.Cell.b0
  Output : Outport
  wires:
  Constant11/1 -> Compare To Constant2/1
  Compare To Constant2/1 -> Switch1/2
  Switch1/1 -> Output/1
  Input/1 -> b0/1, Switch1/3
  a1/1 -> Add1/1
  Add1/1 -> Switch1/1, Unit Delay1/1
  b0/1 -> Add1/2
  Unit Delay1/1 -> a1/1

== system Lib_Piccolo/WOW Archive Container/Load Cell WoW Model 7 - LiftOff Delay variation 4/LPF R ==
  Input : Inport
  Reset : Inport  Port=2
  Add1 : Sum  Inputs=++|
  Compare To Constant2 : simulink/Logic and Bit Operations/Compare To Constant  relop=>  const=0  OutDataTypeStr=uint8
  Constant11 : Constant  Value=Cutoff
  Switch1 : Switch  Criteria=u2 > Threshold
  Unit Delay1 : UnitDelay  InitialCondition=Init  SampleTime=-1
  a1 : Gain  Gain=SensorModel.WOW.Cell.a1
  b0 : Gain  Gain=SensorModel.WOW.Cell.b0
  Output : Outport
  wires:
  Constant11/1 -> Compare To Constant2/1
  Compare To Constant2/1 -> Switch1/2
  Switch1/1 -> Output/1
  Input/1 -> b0/1, Switch1/3
  a1/1 -> Add1/1
  Add1/1 -> Switch1/1, Unit Delay1/1
  b0/1 -> Add1/2
  Unit Delay1/1 -> a1/1

== system Lib_Piccolo/WOW Archive Container/Load Cell WoW Model 7 - LiftOff Delay variation 4/Landing Configuration ==
  Sim.WOW_Filt : Inport
  Piccolo AP Mode : Inport  Port=2
  AND{,1..2,4..5} (5 alike) : Logic  IconShape=distinctive  AllPortsSameDT=off  OutDataTypeStr=boolean
  AND3 : Logic  Inputs=3  IconShape=distinctive  AllPortsSameDT=off  OutDataTypeStr=boolean
  BounceRiskLatch : Subsystem
  BounceRiskTimer : Subsystem  mask{period=SensorModel.WOW.Cell.LiftOffBounceRiskTimeout}
      mask prompts: period "Period [s]"
  Bus Selector : BusSelector  OutputSignals=Sim:WOW_Filt_NG,Sim:WOW_Filt_L,Sim:WOW_Filt_R
  Compare To Constant : simulink/Logic and Bit Operations/Compare To Constant  relop=>  const=9  OutDataTypeStr=boolean
  Compare L : simulink/Logic and Bit Operations/Compare To Constant  relop=>=  const=SensorModel.WOW.Cell.LiftOffBounceRiskThreshold  OutDataTypeStr=boolean
  Compare R1 : simulink/Logic and Bit Operations/Compare To Constant  relop=>=  const=SensorModel.WOW.Cell.LiftOffBounceRiskThreshold  OutDataTypeStr=boolean
  Gain : Gain
  Gain1 : Gain
  Gain2 : Gain
  Hysteresis L : Relay  OnSwitchValue=Ldg_Load_Thresh_Upper  OffSwitchValue=Ldg_Load_Thresh_Lower
  Hysteresis R : Relay  OnSwitchValue=Ldg_Load_Thresh_Upper  OffSwitchValue=Ldg_Load_Thresh_Lower
  LiftOff Double Wheel : Subsystem  mask{period=SensorModel.WOW.Cell.LiftOffLatchTimeDoubleWheel}
      mask prompts: period "Period [s]"
  LiftOff Single Wheel : Subsystem  mask{period=SensorModel.WOW.Cell.LiftOffLatchTimeSingleWheel}
      mask prompts: period "Period [s]"
  NOT{,1..3,5..6} (6 alike) : Logic  Operator=NOT  IconShape=distinctive  AllPortsSameDT=off  OutDataTypeStr=boolean
  OR{,1..3} (4 alike) : Logic  Operator=OR  IconShape=distinctive  AllPortsSameDT=off  OutDataTypeStr=boolean
  Persistance Timer Bounce Risk : Subsystem  mask{period=Ldg_Persist_Time}
      mask prompts: period "Period [s]"
  Persistance Timer Initial Touchdown : Subsystem  mask{period=Ldg_Persist_Time}
      mask prompts: period "Period [s]"
  Terminator : Terminator
  Terminator1 : Terminator
  Terminator2 : Terminator
  Unit Delay : UnitDelay  SampleTime=-1
  detectionLatch : Subsystem
  ContactBool : Outport
  tag scope: BounceRiskActive=global, apModeEnable=global, hasDetected=global
  wires:
  AND3/1 -> OR2/1  "ContactBool-LiftOffPersistanceSingleWheelOff"
  [hasDetected] -> AND4/2, AND3/2
  NOT2/1 -> AND3/1
  AND4/1 -> LiftOff Single Wheel/1(Enable/!Rst)
  NOT/1 -> AND4/1
  OR1/1 -> ContactBool/1  "ContactBool"
  LiftOff Single Wheel/1(Expired) -> NOT2/1  "PersistanceLiftOff"
  Persistance Timer Initial Touchdown/1(Expired) -> detectionLatch/1(D), Gain/1
  Hysteresis L/1 -> OR/1, AND/1, Gain1/1
  Hysteresis R/1 -> OR/2, AND/2, Gain2/1
  Gain1/1 -> Terminator1/1  "ContactL"
  Gain2/1 -> Terminator2/1  "ContactR"
  Gain/1 -> OR1/1  "ContactBool-ActiveContact"
  Sim.WOW_Filt/1 -> Bus Selector/1
  Bus Selector/1 -> Terminator/1  "<Sim:WOW_Filt_NG>"
  Bus Selector/2 -> Compare L/1, Hysteresis L/1  "<Sim:WOW_Filt_L>"
  Bus Selector/3 -> Compare R1/1, Hysteresis R/1  "<Sim:WOW_Filt_R>"
  [apModeEnable] -> AND5/1
  detectionLatch/1(Q_Latched) -> [hasDetected]  "hasDetected"
  Piccolo AP Mode/1 -> Compare To Constant/1
  Compare To Constant/1 -> [apModeEnable]
  LiftOff Double Wheel/1(Expired) -> NOT3/1  "PersistanceLiftOff"
  NOT1/1 -> AND2/1
  [hasDetected] -> AND2/2, AND1/2
  AND1/1 -> OR2/2  "ContactBool-LiftOffPersistanceDoubleWheel"
  NOT3/1 -> AND1/1
  AND2/1 -> LiftOff Double Wheel/1(Enable/!Rst)
  AND/1 -> NOT/1, NOT1/1, Persistance Timer Initial Touchdown/1(Enable/!Rst)
  OR2/1 -> OR1/2  "ContactBool-LiftOffPersistance"
  OR/1 -> AND3/3
  Compare L/1 -> OR3/1
  Compare R1/1 -> OR3/2
  OR3/1 -> Persistance Timer Bounce Risk/1(Enable/!Rst)
  BounceRiskLatch/1(Q_Latched) -> Unit Delay/1, [BounceRiskActive]  "BounceRiskActive"
  NOT5/1 -> BounceRiskLatch/2(Enable/!Rst)
  BounceRiskTimer/1(Expired) -> NOT5/1
  Unit Delay/1 -> BounceRiskTimer/1(Enable/!Rst)
  [BounceRiskActive] -> NOT6/1
  NOT6/1 -> AND5/2
  AND5/1 -> detectionLatch/2(Enable/!Rst)
  Persistance Timer Bounce Risk/1(Expired) -> BounceRiskLatch/1(D)

== system Lib_Piccolo/WOW Archive Container/Load Cell WoW Model 7 - LiftOff Delay variation 4/T//O Configuration ==
  note: Unlike when landing our persistance and latching is inverted relative to Weight Off both gears.
      |
      | Protection against WOW Failure. In the Event of a Sensor Failure and AC lift's off, NZ threshold overides WOW signal.
  Sim.WOW_Filt : Inport
  AND : Logic  IconShape=distinctive  AllPortsSameDT=off  OutDataTypeStr=boolean
  Bus Selector : BusSelector  OutputSignals=Sim:WOW_Filt_NG,Sim:WOW_Filt_L,Sim:WOW_Filt_R
  Compare To Constant1 : simulink/Logic and Bit Operations/Compare To Constant  relop=<  const=TO_Load_Thresh  OutDataTypeStr=uint8
  Compare To Constant2 : simulink/Logic and Bit Operations/Compare To Constant  relop=<  const=TO_Load_Thresh  OutDataTypeStr=uint8
  Latch : Subsystem
  Latch Timer : Subsystem  mask{period=TO_Latch_Time}
      mask prompts: period "Period [s]"
  NOT : Logic  Operator=NOT  IconShape=distinctive  AllPortsSameDT=off  OutDataTypeStr=boolean
  NOT2 : Logic  Operator=NOT  IconShape=distinctive  AllPortsSameDT=off  OutDataTypeStr=boolean
  Persistance Timer : Subsystem  mask{period=TO_Persist_Time}
      mask prompts: period "Period [s]"
  Terminator : Terminator
  Unit Delay : UnitDelay  SampleTime=-1
  ContactBool : Outport
  wires:
  Bus Selector/3 -> Compare To Constant1/1  "<Sim:WOW_Filt_R>"
  Bus Selector/2 -> Compare To Constant2/1  "<Sim:WOW_Filt_L>"
  Bus Selector/1 -> Terminator/1  "<Sim:WOW_Filt_NG>"
  Sim.WOW_Filt/1 -> Bus Selector/1
  NOT/1 -> Latch/2(Enable/!Rst)
  Latch/1(Q_Latched) -> NOT2/1, Unit Delay/1  "ContactBool"
  AND/1 -> Persistance Timer/1(Enable/!Rst)
  Compare To Constant1/1 -> AND/2
  Unit Delay/1 -> Latch Timer/1(Enable/!Rst)
  Latch Timer/1(Expired) -> NOT/1
  Compare To Constant2/1 -> AND/1
  Persistance Timer/1(Expired) -> Latch/1(D)
  NOT2/1 -> ContactBool/1

== system Lib_Piccolo/WOW Archive Container/Load Cell WoW Model 8/Subsystem ==
  note: Ground Detection Logic
  Sim.WOW_NG_N : Inport
  Sim.WOW_L_N : Inport  Port=2
  RESET : Inport  Port=3
  Sim.WOW_R_N : Inport  Port=4
  PICCOLO_AP_MODE : Inport  Port=5
  Bus Creator1 : BusCreator  Inputs=3
  Compare To Constant1 : simulink/Logic and Bit Operations/Compare To Constant  relop===  const=0  OutDataTypeStr=uint8
  Compare To Constant6 : simulink/Logic and Bit Operations/Compare To Constant  relop=>=  const=4  OutDataTypeStr=uint8
  LPF L : Subsystem  mask{Cutoff=SensorModel.WOW.Cell.fc, Init=0}
      mask prompts: Cutoff "Cutoff Frequency [Hz]"; Init "Initial Condition"
  LPF N : Subsystem  mask{Cutoff=SensorModel.WOW.Cell.fc, Init=0}
      mask prompts: Cutoff "Cutoff Frequency [Hz]"; Init "Initial Condition"
  LPF R : Subsystem  mask{Cutoff=SensorModel.WOW.Cell.fc, Init=0}
      mask prompts: Cutoff "Cutoff Frequency [Hz]"; Init "Initial Condition"
  Landing Configuration : Subsystem
  OR : Logic  Operator=OR  IconShape=distinctive  AllPortsSameDT=off  OutDataTypeStr=boolean
  Switch : Switch  Criteria=u2 > Threshold
  T/O Configuration : Subsystem
  Sim.WOW_Filt_NG : Outport
  Sim.WOW_Filt_L : Outport  Port=2
  Contact : Outport  Port=3
  Sim.WOW_Filt_R : Outport  Port=4
  wires:
  Sim.WOW_R_N/1 -> LPF R/1(Input)
  Switch/1 -> Contact/1
  OR/1 -> Switch/2
  T/O Configuration/1(ContactBool) -> Switch/3
  Compare To Constant1/1 -> OR/2
  LPF N/1(Output) -> Bus Creator1/1, Sim.WOW_Filt_NG/1  "Sim.WOW_Filt_NG"
  Landing Configuration/1(ContactBool) -> Switch/1
  Sim.WOW_NG_N/1 -> LPF N/1(Input)
  RESET/1 -> LPF R/2(Reset), LPF L/2(Reset), LPF N/2(Reset)
  Sim.WOW_L_N/1 -> LPF L/1(Input)
  LPF L/1(Output) -> Bus Creator1/2, Sim.WOW_Filt_L/1  "Sim.WOW_Filt_L"
  Bus Creator1/1 -> Landing Configuration/1(Sim.WOW_Filt), T/O Configuration/1(Sim.WOW_Filt)
  Compare To Constant6/1 -> OR/1
  PICCOLO_AP_MODE/1 -> Compare To Constant6/1, Compare To Constant1/1
  LPF R/1(Output) -> Bus Creator1/3, Sim.WOW_Filt_R/1  "Sim.WOW_Filt_R"
